simulink model "structure_impl_mower"  (R2026b)
settings: Solver=VariableStepAuto
undefined symbols (not defined in the file or in its folder): DiscIntNeverNeededParam, P, Ts
libraries: fl_lib x9, nesl_utility x5, simulink x2
settings Model: Creator=aomar  LastModifiedBy=aomar

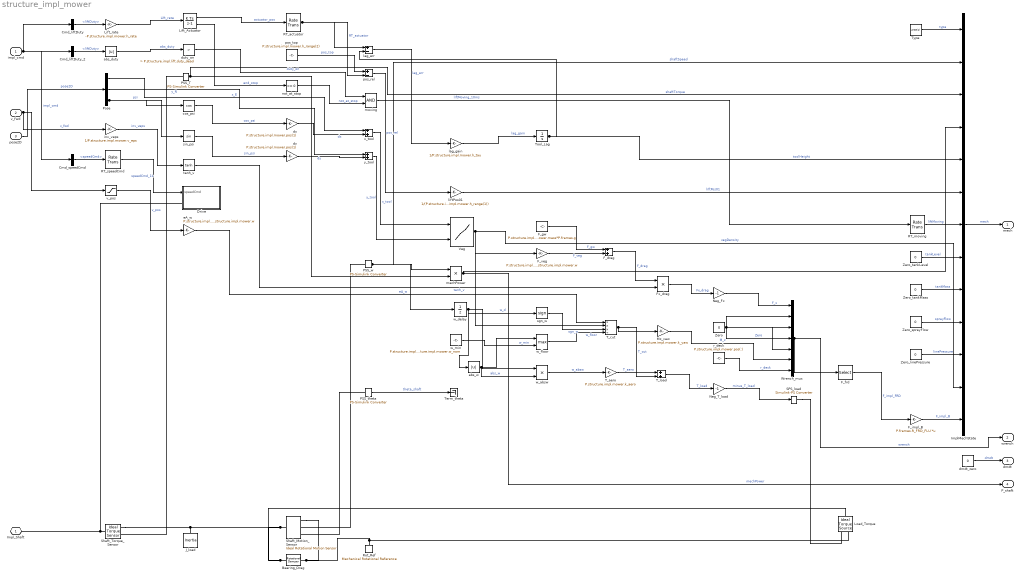
== system structure_impl_mower ==
  impl_cmd : Inport  OutDataTypeStr=Bus: Bus_ImplementCmd  SampleTime=Ts.ctrl
  v_fwd : Inport  Port=2
  pose2D : Inport  Port=3
  Bearing_Drag : fl_lib/Mechanical/Rotational Elements/Rotational Damper  D=P.structure.impl.mower.D N*m*s/rad  w_specify=off  w_priority=None  w=0 rad/s  w_nominal_specify=off  w_nominal_value=1  w_nominal_unit=rad/s  t_specify=off  t_priority=None  t=0 N*m  t_nominal_specify=off  t_nominal_value=1  t_nominal_unit=N*m
  Cmd_liftDuty : BusSelector  OutputSignals=liftDuty
  Cmd_liftDuty_2 : BusSelector  OutputSignals=liftDuty
  Cmd_speedCmd : BusSelector  OutputSignals=speedCmd
  Drive : Subsystem  Variant=on
  F_drag : Sum
  F_frd : Selector  InputPortWidth=9  IndexOptions=Index vector (dialog)  Indices=1:3  OutputSizes=1
  F_gw : Constant  Value=P.structure.impl.mower.f_gw*P.structure.impl.mower.lambda_gw*P.structure.impl.mower.mass*P.frames.g  VectorParams1D=off
  F_impl_B : Gain  Gain=P.frames.R_FRD_FLU  Multiplication=Matrix(K*u)
  F_veg : Gain  Gain=P.structure.impl.mower.c_veg*P.structure.impl.mower.w
  Fx_drag : Product  Inputs=**
  ImplMechState : BusCreator  Inputs=13  OutDataTypeStr=Bus: Bus_ImplMechState  NonVirtualBus=on
  J_load : fl_lib/Mechanical/Rotational Elements/Inertia  inertia=P.structure.impl.mower.J kg*m^2  num_ports=foundation.enum.numPorts2.one  w_specify=off  w_priority=High  w=0 rad/s  w_nominal_specify=off  w_nominal_value=1  w_nominal_unit=rad/s  t_specify=off  t_priority=None  t=0 N*m  t_nominal_specify=off  t_nominal_value=1  t_nominal_unit=N*m
  Lift_Actuator : DiscreteIntegrator  gainval=1  InitialCondition=P.structure.impl.mower.h0  SampleTime=Ts.ctrl  LimitOutput=on  UpperSaturationLimit=P.structure.impl.mower.h_range(2)  LowerSaturationLimit=P.structure.impl.mower.h_range(1)  ShowSaturationPort=on  ICPrevOutput=DiscIntNeverNeededParam  ICPrevScaledInput=DiscIntNeverNeededParam
  Lift_rate : Gain  Gain=-P.structure.impl.mower.h_rate
  Load_Torque : fl_lib/Mechanical/Mechanical Sources/Ideal Torque Source
  Mz_yaw : Gain  Gain=P.structure.impl.mower.k_yaw
  Neg_Fx : Gain  Gain=-1
  Neg_T_load : Gain  Gain=-1
  PSS_T : nesl_utility/PS-Simulink Converter  PhysicalDomain=network_engine_domain  SubClassName=ps_output  LeftPortType=input  RightPortType=output  PseudoPeriodic=off  Frequencies=[]  VectorFormat=inherit  Unit=N*m  AffineConversion=off
  PSS_theta : nesl_utility/PS-Simulink Converter  PhysicalDomain=network_engine_domain  SubClassName=ps_output  LeftPortType=input  RightPortType=output  PseudoPeriodic=off  Frequencies=[]  VectorFormat=inherit  Unit=rad  AffineConversion=off
  PSS_w : nesl_utility/PS-Simulink Converter  PhysicalDomain=network_engine_domain  SubClassName=ps_output  LeftPortType=input  RightPortType=output  PseudoPeriodic=off  Frequencies=[]  VectorFormat=inherit  Unit=rad/s  AffineConversion=off
  Pose : Demux  Outputs=3
  RT_actuator : RateTransition  InitialCondition=P.structure.impl.mower.h0  OutPortSampleTime=Ts.base
  RT_moving : RateTransition  InitialCondition=false  OutPortSampleTime=Ts.base
  RT_speedCmd : RateTransition  OutPortSampleTime=Ts.base
  Rot_Ref : fl_lib/Mechanical/Rotational Elements/Mechanical Rotational Reference
  SPS_load : nesl_utility/Simulink-PS Converter  PhysicalDomain=network_engine_domain  SubClassName=ps_input  LeftPortType=input  RightPortType=output  PseudoPeriodic=off  Frequencies=[]  NoiseDistribution=none  NoiseParameters=[]  Unit=N*m  AffineConversion=off  FilteringAndDerivatives=zero  SimscapeFilterOrder=1  InputFilterTimeConstant=0.001  UdotUserProvided=0
  Shaft_Motion_Sensor : fl_lib/Mechanical/Mechanical Sensors/Ideal Rotational Motion Sensor  reference=foundation.enum.MeasurementReference.difference  acceleration_port=false  velocity_port=true  position_port=true  wrap_angle=false  offset=0 rad
  Shaft_Torque_Sensor : fl_lib/Mechanical/Mechanical Sensors/Ideal Torque Sensor
  T_aero : Gain  Gain=P.structure.impl.mower.k_aero
  T_cut : Product  Inputs=***/
  T_load : Sum
  Term_theta : Terminator
  Tool_Lag : Integrator  InitialCondition=P.structure.impl.mower.h0
  Type : Constant  Value=uint8(1)  VectorParams1D=off  OutDataTypeStr=uint8
  Veg : Lookup_n-D  BreakpointsForDimension1=P.world.terrain.xE  BreakpointsForDimension2=P.world.terrain.yN  IndexSearchMethod=Evenly spaced points  Table=P.world.veg.rho  ExtrapMethod=Clip  InternalRulePriority=Speed  RndMeth=Simplest
      settings: InputPortMap=u0,u1
  Wrench_mux : Mux  Inputs=7
  Zero : Constant  Value=0  VectorParams1D=off
  Zero_linePressure : Constant  Value=0  VectorParams1D=off
  Zero_sprayFlow : Constant  Value=0  VectorParams1D=off
  Zero_tankLevel : Constant  Value=0  VectorParams1D=off
  Zero_tankMass : Constant  Value=0  VectorParams1D=off
  abs_duty : Abs  ZeroCross=off  SaturateOnIntegerOverflow=off
  abs_w : Abs  ZeroCross=off  SaturateOnIntegerOverflow=off
  cos_psi : Trigonometry  Operator=cos
  dmdt_zero : Constant  Value=0  VectorParams1D=off
  duty_on : simulink/Logic and Bit Operations/Compare To Constant  relop=>  const=P.structure.impl.lift.duty_dead  OutDataTypeStr=boolean
  dx : Gain  Gain=P.structure.impl.mower.pos(1)
  dy : Gain  Gain=P.structure.impl.mower.pos(1)
  eA_w : Gain  Gain=P.structure.impl.mower.e_A*P.structure.impl.mower.w
  inv_veps : Gain  Gain=1/P.structure.impl.mower.v_eps
  lag_err : Sum  Inputs=+-
  lag_gain : Gain  Gain=1/P.structure.impl.mower.h_tau
  liftPos01 : Gain  Gain=1/(P.structure.impl.mower.h_range(2)-P.structure.impl.mower.h_range(1))
  mechPower : Product  Inputs=**
  moving : Logic  AllPortsSameDT=off  OutDataTypeStr=boolean
  not_at_stop : simulink/Logic and Bit Operations/Compare To Zero  relop===  OutDataTypeStr=boolean
  pos_rel : Sum  Inputs=+-
  pos_top : Constant  Value=P.structure.impl.mower.h_range(2)  VectorParams1D=off
  r_deck : Constant  Value=P.structure.impl.mower.pos(:)  VectorParams1D=off
  sgn_w : Signum  ZeroCross=off
  sin_psi : Trigonometry
  tanh_v : Trigonometry  Operator=tanh
  v_pos : Saturate  UpperLimit=inf  LowerLimit=0
  w_absw : Product  Inputs=**
  w_delay : UnitDelay  SampleTime=Ts.base
  w_floor : MinMax  Function=max  Inputs=2  ZeroCross=off
  w_min : Constant  Value=P.structure.impl.mower.w_min_frac*P.structure.impl.mower.w_nom  VectorParams1D=off
  x_tool : Sum
  y_tool : Sum
  Impl_Shaft : PMIOPort  Side=Left  ConnectionType=Connection: foundation.mechanical.rotational.rotational
  mech : Outport  OutDataTypeStr=Bus: Bus_ImplMechState
  wrench : Outport  Port=2
  dmdt : Outport  Port=3
  P_shaft : Outport  Port=4
  wires:
  impl_cmd/1 -> Cmd_speedCmd/1, Cmd_liftDuty/1, Cmd_liftDuty_2/1  "impl_cmd"
  v_fwd/1 -> v_pos/1, inv_veps/1  "v_fwd"
  pose2D/1 -> Pose/1  "pose2D"
  Cmd_liftDuty/1 -> Lift_rate/1  "<liftDuty>"
  Cmd_liftDuty_2/1 -> abs_duty/1  "<liftDuty>"
  Cmd_speedCmd/1 -> RT_speedCmd/1  "<speedCmd>"
  Pose/1 -> x_tool/1  "x_E"
  Pose/2 -> y_tool/1  "y_N"
  Pose/3 -> sin_psi/1, cos_psi/1  "psi"
  Lift_rate/1 -> Lift_Actuator/1  "Lift_rate"
  abs_duty/1 -> duty_on/1  "abs_duty"
  inv_veps/1 -> tanh_v/1  "inv_veps"
  v_pos/1 -> eA_w/1  "v_pos"
  RT_speedCmd/1 -> Drive/1(speedCmd)  "speedCmd_1k"
  PSS_T/1 -> mechPower/2, ImplMechState/3  "shaftTorque"
  duty_on/1 -> moving/1  "duty_on"
  cos_psi/1 -> dx/1  "cos_psi"
  sin_psi/1 -> dy/1  "sin_psi"
  tanh_v/1 -> Fx_drag/2  "tanh_v"
  eA_w/1 -> T_cut/1  "eA_w"
  Lift_Actuator/1 -> RT_actuator/1  "actuator_pos"
  Lift_Actuator/2 -> not_at_stop/1  "end_stop"
  pos_top/1 -> pos_rel/1  "pos_top"
  not_at_stop/1 -> moving/2  "not_at_stop"
  dx/1 -> x_tool/2  "dx"
  dy/1 -> y_tool/2  "dy"
  RT_actuator/1 -> pos_rel/2, lag_err/1  "RT_actuator"
  PSS_w/1 -> ImplMechState/2, w_delay/1, mechPower/1  "shaftSpeed"
  PSS_theta/1 -> Term_theta/1  "theta_shaft"
  lag_err/1 -> lag_gain/1  "lag_err"
  pos_rel/1 -> liftPos01/1  "pos_rel"
  x_tool/1 -> Veg/1  "x_tool"
  y_tool/1 -> Veg/2  "y_tool"
  moving/1 -> RT_moving/1  "liftMoving_10ms"
  lag_gain/1 -> Tool_Lag/1  "lag_gain"
  liftPos01/1 -> ImplMechState/6  "liftPos01"
  mechPower/1 -> P_shaft/1, ImplMechState/4  "mechPower"
  w_min/1 -> w_floor/2  "w_min"
  w_delay/1 -> w_absw/1, abs_w/1, sgn_w/1  "w_d"
  Veg/1 -> ImplMechState/12, T_cut/2, F_veg/1  "vegDensity"
  abs_w/1 -> w_floor/1, w_absw/2  "abs_w"
  Tool_Lag/1 -> lag_err/2, ImplMechState/5  "toolHeight"
  F_gw/1 -> F_drag/1  "F_gw"
  F_veg/1 -> F_drag/2  "F_veg"
  sgn_w/1 -> T_cut/3  "sgn_w"
  w_floor/1 -> T_cut/4  "w_floor"
  w_absw/1 -> T_aero/1  "w_absw"
  F_drag/1 -> Fx_drag/1  "F_drag"
  T_cut/1 -> T_load/2, Mz_yaw/1  "T_cut"
  T_aero/1 -> T_load/1  "T_aero"
  T_load/1 -> Neg_T_load/1  "T_load"
  Fx_drag/1 -> Neg_Fx/1  "Fx_drag"
  Mz_yaw/1 -> Wrench_mux/6  "M_z"
  Neg_Fx/1 -> Wrench_mux/1  "F_x"
  Zero/1 -> Wrench_mux/5, Wrench_mux/2, Wrench_mux/4, Wrench_mux/3  "Zero"
  r_deck/1 -> Wrench_mux/7  "r_deck"
  Neg_T_load/1 -> SPS_load/1  "minus_T_load"
  Wrench_mux/1 -> wrench/1, F_frd/1  "wrench"
  F_frd/1 -> F_impl_B/1  "F_impl_FRD"
  Type/1 -> ImplMechState/1  "type"
  Zero_tankLevel/1 -> ImplMechState/8  "tankLevel"
  Zero_tankMass/1 -> ImplMechState/9  "tankMass"
  Zero_sprayFlow/1 -> ImplMechState/10  "sprayFlow"
  Zero_linePressure/1 -> ImplMechState/11  "linePressure"
  F_impl_B/1 -> ImplMechState/13  "F_impl_B"
  RT_moving/1 -> ImplMechState/7  "liftMoving"
  ImplMechState/1 -> mech/1  "mech"
  dmdt_zero/1 -> dmdt/1  "dmdt"
  connections:
  J_load/LConn1 -- Shaft_Torque_Sensor/RConn1 -- Shaft_Motion_Sensor/LConn1 -- Bearing_Drag/LConn1 -- Load_Torque/LConn1
  Bearing_Drag/RConn1 -- Shaft_Motion_Sensor/RConn1 -- Rot_Ref/LConn1 -- Load_Torque/RConn2
  Shaft_Torque_Sensor/LConn1 -- Drive/LConn1 -- Impl_Shaft/RConn1
  SPS_load/RConn1 -- Load_Torque/RConn1
  PSS_T/LConn1 -- Shaft_Torque_Sensor/RConn2
  PSS_theta/LConn1 -- Shaft_Motion_Sensor/RConn3
  PSS_w/LConn1 -- Shaft_Motion_Sensor/RConn2

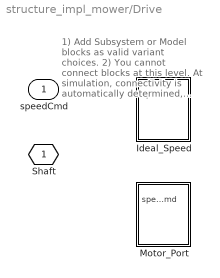
== system structure_impl_mower/Drive ==
  note: 1) Add Subsystem or Model blocks as valid variant choices.
      | 2) You cannot connect blocks at this level. At simulation, connectivity is automatically
      | determined, based on the active variant and port name matching.
  speedCmd : Inport
  Ideal_Speed : Subsystem  VariantControl=VC_IMPL_DRIVE == 1
  Motor_Port : Subsystem  VariantControl=VC_IMPL_DRIVE == 2
  Shaft : PMIOPort  Side=Left  ConnectionType=Connection: foundation.mechanical.rotational.rotational

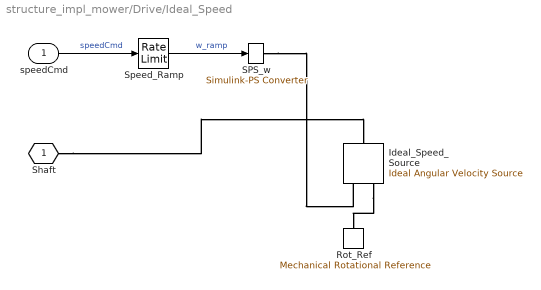
== system structure_impl_mower/Drive/Ideal_Speed ==
  speedCmd : Inport
  Ideal_Speed_Source : fl_lib/Mechanical/Mechanical Sources/Ideal Angular Velocity Source
  Rot_Ref : fl_lib/Mechanical/Rotational Elements/Mechanical Rotational Reference
  SPS_w : nesl_utility/Simulink-PS Converter  PhysicalDomain=network_engine_domain  SubClassName=ps_input  LeftPortType=input  RightPortType=output  PseudoPeriodic=off  Frequencies=[]  NoiseDistribution=none  NoiseParameters=[]  Unit=rad/s  AffineConversion=off  FilteringAndDerivatives=filter  SimscapeFilterOrder=1  InputFilterTimeConstant=P.structure.impl.drive.tau_f  UdotUserProvided=0
  Speed_Ramp : RateLimiter  RisingSlewLimit=P.structure.impl.drive.a_max  FallingSlewLimit=-P.structure.impl.drive.a_max  SampleTimeMode=inherited
  Shaft : PMIOPort  Side=Left  ConnectionType=Connection: foundation.mechanical.rotational.rotational
  wires:
  speedCmd/1 -> Speed_Ramp/1  "speedCmd"
  Speed_Ramp/1 -> SPS_w/1  "w_ramp"
  connections:
  Shaft/RConn1 -- Ideal_Speed_Source/LConn1
  SPS_w/RConn1 -- Ideal_Speed_Source/RConn1
  Ideal_Speed_Source/RConn2 -- Rot_Ref/LConn1

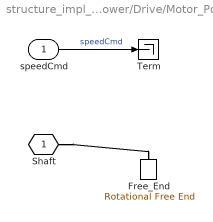
== system structure_impl_mower/Drive/Motor_Port ==
  speedCmd : Inport
  Free_End : fl_lib/Mechanical/Rotational Elements/Rotational Free End  w_specify=off  w_priority=None  w=0 rad/s  w_nominal_specify=off  w_nominal_value=1  w_nominal_unit=rad/s
  Term : Terminator
  Shaft : PMIOPort  Side=Left  ConnectionType=Connection: foundation.mechanical.rotational.rotational
  wires:
  speedCmd/1 -> Term/1  "speedCmd"
  connections:
  Shaft/RConn1 -- Free_End/LConn1
